simulink model "pmsm_cc"  (R2023b)
settings: Solver=FixedStepDiscrete  StartTime=0.0  StopTime=0.6  FixedStep=1e-5  RelTol=1e-3
values from neighbouring files (symbols this model uses):
  V = out.flog.signals.values    [add_ident2.m]    (also in add_w.m; add_w2.m; baseline_model.m; check_kt.m = out.mlog.signals.values)
libraries: spsControlledVoltageSourceLib x3, spsPermanentMagnetSynchronousMachineLib x1, spspowerguiLib x1
settings Model: Creator=28447  LastModifiedBy=28447

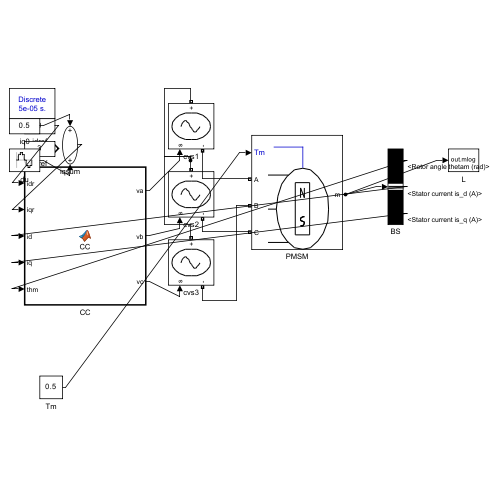
[thumbnail: Simulink's stored preview of the top-level diagram]
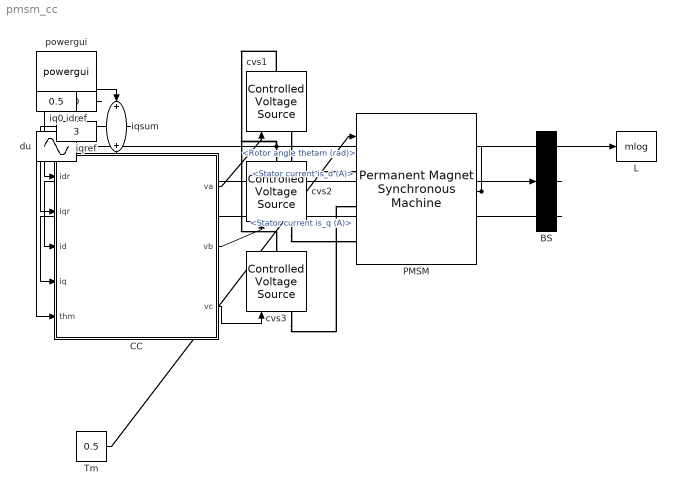
== system pmsm_cc ==
  BS : BusSelector  OutputSignals=Rotor angle thetam (rad),Stator current is_d (A),Stator current is_q (A)
  CC : MATLAB Function  TreatAsAtomicUnit=on
  L : ToWorkspace  VariableName=mlog  SaveFormat=Structure With Time  SampleTime=-1
  PMSM : spsPermanentMagnetSynchronousMachineLib/Permanent Magnet Synchronous Machine  NbPhases=3  FluxDistribution=Sinusoidal  RotorType=Round  MechanicalLoad=Torque Tm  PresetModel=No  ShowDetailedParameters=on  MeasurementBus=off  Resistance=0.175  Inductance=0.57e-3  dqInductances=[8.5e-3,8.5e-3]  La=0.000395  MachineConstant=Flux linkage established by magnets (V.s)  Flux=0.016833  VoltageCst=12.2127  TorqueCst=0.101  Flat=120  Mechanical=[1.89e-5 0 4 0]  PolePairs=4  InitialConditions=[0,0, 0,0]  InitialConditions5ph=[0 0 0 0 0 0]  RefAngle=90 degrees behind phase A axis (modified Park)  IterativeDiscreteModel=Trapezoidal non iterative  TsBlock=-1  TsPowergui=0
  Tm : Constant  Value=0.5
  cvs1 : spsControlledVoltageSourceLib/Controlled Voltage Source  Initialize=on  Source_Type=AC  Amplitude=0  Phase=0  Frequency=0  Measurements=None
  cvs2 : spsControlledVoltageSourceLib/Controlled Voltage Source  Initialize=on  Source_Type=AC  Amplitude=0  Phase=0  Frequency=0  Measurements=None
  cvs3 : spsControlledVoltageSourceLib/Controlled Voltage Source  Initialize=on  Source_Type=AC  Amplitude=0  Phase=0  Frequency=0  Measurements=None
  du : Sin  Amplitude=0.118  Frequency=2*pi*65  SampleTime=5e-5
  idref : Constant  Value=0
  iq0 : Constant  Value=0.5
  iqref : Constant  Value=3
  iqsum : Sum
  powergui : spspowerguiLib/powergui  Priority=1  SimulationMode=Discrete  SampleTime=50e-6  frequency=60  Iterations=50  frequencyindice=60  Pbase=100e6  ErrMax=1e-4  UnitsV=kV  UnitsW=MW  buscounter=0  FunctionMessages=off  echomessages=off  EnableUseOfTLC=off  CurrentSourceSwitches=off  DisableSnubberDevices=off  DisableRonSwitches=off  DisableVfSwitches=off  DisplayEquations=off  AutomaticDiscreteSolvers=off  SolverType=Tustin/Backward Euler (TBE)  Interpol=off  ExternalGateDelay=off  methode=off  Ts=1e-5  x0status=blocks  SPID=on  SwTol=0  HookPort=off  NonlinearTolerance=1e-4  nMaxIteration=100  ContinueOnMaxIteration=off  RestoreLinks=warning  ResistiveCurrentMeasurement=off  Frange=[0:2:500]  Ylog=off  Xlog=on  ShowGrid=off  save=off  variable=ZData  structure=0  ZoomFFT=off  StartTime=0.0  cycles=1  DisplayStyle=1  fundamental=60  FreqAxis=off  MaxFrequency=1000  frequencyindicesteady=1  RmsSteady=1  display=off
  wires:
  Tm/1 -> PMSM/1
  PMSM/1 -> BS/1, L/1
  idref/1 -> CC/1(idr)
  BS/2 -> CC/3(id)  "<Stator current is_d (A)>"
  BS/3 -> CC/4(iq)  "<Stator current is_q (A)>"
  BS/1 -> CC/5(thm)  "<Rotor angle thetam (rad)>"
  CC/1(va) -> cvs1/1
  CC/2(vb) -> cvs2/1
  CC/3(vc) -> cvs3/1
  iq0/1 -> iqsum/1
  du/1 -> iqsum/2
  iqsum/1 -> CC/2(iqr)
  connections:
  cvs1/LConn1 -- PMSM/LConn1
  cvs2/LConn1 -- PMSM/LConn2
  cvs3/LConn1 -- PMSM/LConn3
  cvs2/RConn1 -- cvs1/RConn1 -- cvs3/RConn1

== matlab function pmsm_cc/CC ==
  data: idr input; va output; iqr input; id input; iq input; thm input; vb output; vc output
function [va, vb, vc] = CC(idr, iqr, id, iq, thm)
% 电流环 20 kHz（Ts=5e-5）+ 反 Park
% 标定结果（2026-11-24，静止注入扫描）：机器 d 轴在 phase-A 轴 +90° 处
%   phi=90° 时 id=V/R、iq≈0  =>  theta_e = p*thm + pi/2
persistent xi xq
Ts = 5e-5; p = 4;
Kp = 7.2; Ki = 2200;
if isempty(xi), xi = 0; xq = 0; end
ed = idr - id;
eq = iqr - iq;
xi = xi + Ki*Ts*ed;
xq = xq + Ki*Ts*eq;
vd = Kp*ed + xi;
vq = Kp*eq + xq;
th = p*thm + pi/2;
va = vd*cos(th) - vq*sin(th);
vb = vd*cos(th - 2*pi/3) - vq*sin(th - 2*pi/3);
vc = vd*cos(th + 2*pi/3) - vq*sin(th + 2*pi/3);
end
